simulink model "PAM"  (R2016a)
settings: Solver=VariableStepAuto  StartTime=0.0  StopTime=10.0  RelTol=1e-3
settings Model: Creator=T H Mahir  LastModifiedBy=T H Mahir

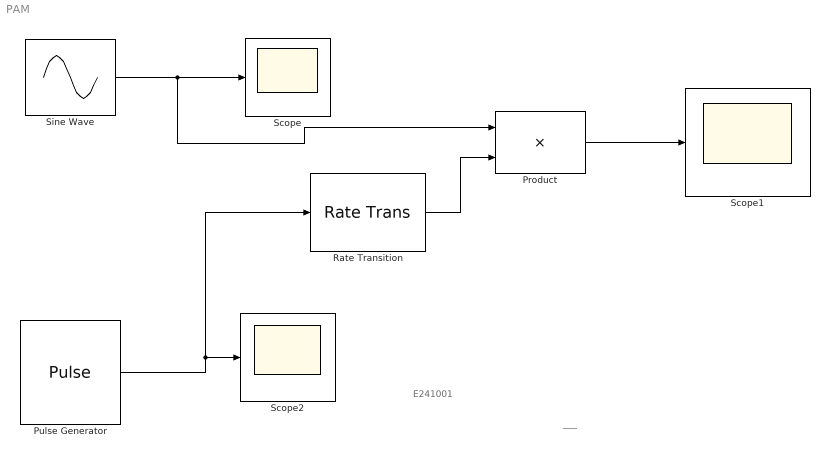
== system PAM ==
  note: E241001
  note: ___
  Product : Product
  Pulse Generator : DiscretePulseGenerator  PulseType=Time based  Period=0.2  PulseWidth=20
  Rate Transition : RateTransition
  Scope : Scope
  Scope1 : Scope
  Scope2 : Scope
  Sine Wave : Sin  Amplitude=5  Phase=0.01  SampleTime=0
  wires:
  Pulse Generator/1 -> Rate Transition/1, Scope2/1
  Sine Wave/1 -> Product/1, Scope/1
  Rate Transition/1 -> Product/2
  Product/1 -> Scope1/1
